simulink model "My_gfm_battery_sil_12_ConvIGBT_zDomain"  (R2025b)
settings: Solver=ode23t  StartTime=0.0  StopTime=10  MaxStep=1e-4  RelTol=1e-3
PreLoadFcn:
  | close all;
  | clear all;
  | clc;
  | 
  | 
  | modelDir = fileparts(get_param(bdroot,'FileName'));
  | 
  | load_system(fullfile(modelDir,'controls_element_lib.slx'));
  | load_system(fullfile(modelDir,'test_sequence_lib.slx'));
  | 
  | Simulink.importExternalCTypes('.\circuitControls\circuitControls_A_autogen.h')
InitFcn:
  | % frequency nominals
  | F_NOM = 60;
  | W_NOM = 2 * pi * F_NOM;
  | 
  | % base values relative to inverter
  | % --------------------------------
  | VLL_INV_NOM = 480;
  | P_INV_NOM = 1e6;
  | Q_INV_NOM = 0.5e6;
  | S_INV_NOM = sqrt(P_INV_NOM^2 + Q_INV_NOM^2);
  | 
  | I_INV_BASE = S_INV_NOM/(sqrt(3)*VLL_INV_NOM);
  | Z_INV_BASE = VLL_INV_NOM^2/S_INV_NOM;
  | L_INV_BASE = Z_INV_BASE / W_NOM;
  | C_INV_BASE = 1 / (Z_INV_BASE * W_NOM);
  | 
  | % nominal ratings for power system model
  | % --------------------------------------
  | INVERTER_COUNT = 100;
  | 
  | VLV_NOM = VLL_INV_NOM;
  | VMV_NOM = 35e3;
  | VHV_NOM = 230e3;
  | S_PLANT = INVERTER_COUNT * S_INV_NOM;
  | 
  | N_GSU = VHV_NOM/VMV_NOM;
  | N_MVT = VMV_NOM/VLV_NOM;
  | 
  | I_LV_BASE = S_PLANT/(sqrt(3)*VLV_NOM);
  | I_MV_BASE = S_PLANT/(sqrt(3)*VMV_NOM);
  | I_HV_BASE = S_PLANT/(sqrt(3)*VHV_NOM);
  | 
  | Z_LV_BASE = VLV_NOM^2/S_PLANT;
  | Z_MV_BASE = VMV_NOM^2/S_PLANT;
  | Z_HV_BASE = VHV_NOM^2/S_PLANT;
  | 
  | L_LV_BASE = Z_LV_BASE / W_NOM;
  | L_MV_BASE = Z_MV_BASE / W_NOM;
  | L_HV_BASE = Z_HV_BASE / W_NOM;
  | C_LV_BASE = 1 / (Z_LV_BASE * W_NOM);
  | C_MV_BASE = 1 / (Z_MV_BASE * W_NOM);
  | C_HV_BASE = 1 / (Z_HV_BASE * W_NOM);
undefined symbols (not defined in the file): D1, D11, Delta, gcbh, j, SampleTime, sps_rtmsupport, Ts
libraries: simulink x56, spsVoltageMeasurementLib x21, spsThreePhaseSeriesRLCBranchLib x20, spsControlledCurrentSourceLib x20, spsControlledVoltageSourceLib x15, spsThreePhaseVIMeasurementLib x12, spsSeriesRLCBranchLib x11, spsGroundLib x11, test_sequence_lib x10, controls_element_lib x8, spsCurrentMeasurementLib x8, spsThreePhaseTransformerTwoWindingsLib x6
(part 9 of 9)

== system My_gfm_battery_sil_12_ConvIGBT_zDomain/My Inverter Controller /My_machineModel_A1/governer1/LPF(DamperDecoupler) limited 1 ==
  In : Inport
  1/tau_damp : Gain  Gain=1/0.3
  Integrator : Integrator  LimitOutput=on  UpperSaturationLimit=1.2*SRated  LowerSaturationLimit=-1.2*SRated
  Sum3 : Sum  Inputs=|+-
  Out : Outport
  wires:
  Integrator/1 -> Out/1, Sum3/2
  Sum3/1 -> 1/tau_damp/1
  In/1 -> Sum3/1
  1/tau_damp/1 -> Integrator/1

== system My_gfm_battery_sil_12_ConvIGBT_zDomain/My Inverter Controller /My_machineModel_A1/governer1/synchronizer ==
  note: Why?
  note: Big Range?
  note: prevent it from acting during typical faults
  note: Prevent loss of sync at low voltage events, using asym filter to traget long extended low voltage events
  note: Keeps the machine spining in synchronize while machine is disabled, disabling the machine means
  note: Why?
  note: Should be sqrt(Vd^2 + Vq^2) ?
  Vq : Inport
  Vd : Inport  Port=2
  machine_enabled : Inport  Port=3
  Constant : Constant
  Gain : Gain  Gain=SRated
  Gain2 : Gain  Gain=1/VllRated
  HPF : Subsystem
  Product1 : Product
  Saturation : Saturate  UpperLimit=1  LowerLimit=0
  Sum : Sum  Inputs=|++
  Sum2 : Sum  Inputs=|+-
  Switch : Switch  Criteria=u2 > Threshold  SaturateOnIntegerOverflow=off  InputSameDT=off
  Transfer Fcn : TransferFcn  Commented=on  Numerator=[(2 * pi * 50) 0]  Denominator=[1, (2*pi*50)]
  assymmetric filter1 : Subsystem
  gain : Gain  Gain=2*pi*50
  kFastSync : Gain
  kSync : Gain  Gain=20
  pSyncLimit : Saturate  UpperLimit=3  LowerLimit=-3
  syncFadeGain : Gain  Gain=4
  syncFadeThreshold : Constant  Value=0.2
  to_pu : Gain  Gain=1 / VllRated
  p_sync_pu : Outport
  wires:
  to_pu/1 -> Sum2/2
  Vd/1 -> assymmetric filter1/1(in)
  assymmetric filter1/1(out) -> to_pu/1
  pSyncLimit/1 -> Gain/1
  kSync/1 -> Sum/1
  Sum/1 -> pSyncLimit/1
  Product1/1 -> p_sync_pu/1
  Constant/1 -> Switch/3
  Sum2/1 -> syncFadeGain/1
  machine_enabled/1 -> Switch/2
  syncFadeGain/1 -> Saturation/1
  Saturation/1 -> Switch/1
  syncFadeThreshold/1 -> Sum2/1
  Switch/1 -> Product1/2
  Gain2/1 -> kFastSync/1, kSync/1
  Vq/1 -> Gain2/1
  Gain/1 -> Product1/1  "p_sync"
  kFastSync/1 -> HPF/1(in)
  HPF/1(out) -> gain/1
  gain/1 -> Sum/2

== system My_gfm_battery_sil_12_ConvIGBT_zDomain/My Inverter Controller /My_machineModel_A1/rotor model/HPF (wDamperDecoupler) 1 ==
  in : Inport
  1/tau_damp : Gain  Gain=1/0.3
  Integrator : Integrator
  Sum : Sum  Inputs=|+-
  out : Outport
  wires:
  Sum/1 -> out/1, 1/tau_damp/1
  in/1 -> Sum/1
  Integrator/1 -> Sum/2
  1/tau_damp/1 -> Integrator/1

== system My_gfm_battery_sil_12_ConvIGBT_zDomain/My Inverter Controller /My_machineModel_A1/rotor model/oscillator_3ph ==
  f : Inport
  Cos : Trigonometry  Operator=cos
  Gain : Gain  Gain=2*pi
  Integrator : Integrator
  Real-Imag to Complex : RealImagToComplex
  Sin : Trigonometry
  Sum1 : Sum  Inputs=|++
  phase_shift : Constant  Value=[0 -1/3 -2/3]
  osc[3] : Outport
  wires:
  f/1 -> Integrator/1
  Real-Imag to Complex/1 -> osc[3]/1
  Cos/1 -> Real-Imag to Complex/1
  Gain/1 -> Cos/1, Sin/1
  Integrator/1 -> Sum1/1
  Sin/1 -> Real-Imag to Complex/2
  phase_shift/1 -> Sum1/2
  Sum1/1 -> Gain/1

== system My_gfm_battery_sil_12_ConvIGBT_zDomain/My Inverter Controller /My_machineModel_Other Exciter/AVR/Asym filter ==
  note: Forward integrator
  in : Inport
  Constant : Constant  Value=Ts
  Constant1 : Constant  Value=Ts
  Constant2 : Constant  Value=OmegaUp
  Constant3 : Constant  Value=OmegaUp
  Constant4 : Constant  Value=OmegaDn
  Delay : Delay  DelayLength=1  InitialCondition=0
  Product{,1..4} (5 alike) : Product
  Saturation : Saturate  UpperLimit=inf  LowerLimit=0
  Saturation1 : Saturate  UpperLimit=0  LowerLimit=-inf
  Sum : Sum  Inputs=|++
  Sum1 : Sum  Inputs=|++
  Sum4 : Sum  Inputs=|+-
  out : Outport
  wires:
  Delay/1 -> Sum4/2, Sum/2
  in/1 -> Sum4/1, Product4/2
  Sum4/1 -> Product2/1, Product1/2
  Sum/1 -> out/1, Delay/1
  Saturation/1 -> Sum1/1
  Saturation1/1 -> Sum1/2
  Sum1/1 -> Product/2
  Product/1 -> Sum/1
  Constant/1 -> Product/1
  Constant3/1 -> Product1/1
  Constant4/1 -> Product2/2
  Product1/1 -> Saturation/1
  Product2/1 -> Saturation1/1
  Product4/1 -> Product3/2
  Constant1/1 -> Product3/1
  Constant2/1 -> Product4/1

== system My_gfm_battery_sil_12_ConvIGBT_zDomain/My Inverter Controller /My_machineModel_Other Exciter/AVR/Integrator1 ==
  in : Inport
  rst : Inport  Port=2
  Constant : Constant  Value=0
  Constant1 : Constant  Value=HiLim
  Constant2 : Constant  Value=LoLim
  Constant3 : Constant  Value=Ts
  Delay : Delay  DelayLength=1  InitialCondition=0
  Logical Operator : Logic  Operator=NOT  AllPortsSameDT=off  OutDataTypeStr=boolean
  Product : Product
  Saturation Dynamic : simulink/Discontinuities/Saturation Dynamic  OutMin=[]  OutMax=[]  OutDataTypeStr=Inherit: Same as second input  OutDataType=fixdt(1, 16)  OutScaling=2^-10  DoSatur=off
  Sum : Sum  Inputs=|++
  Switch : Switch  Criteria=u2 ~= 0  SaturateOnIntegerOverflow=off  InputSameDT=off
  out : Outport
  FB : Outport  Port=2
  wires:
  Delay/1 -> Sum/2, FB/1
  Switch/1 -> Saturation Dynamic/2
  in/1 -> Product/2
  Product/1 -> Sum/1
  Constant3/1 -> Product/1
  Sum/1 -> Switch/1
  Constant/1 -> Switch/3
  rst/1 -> Logical Operator/1
  Logical Operator/1 -> Switch/2
  Saturation Dynamic/1 -> out/1, Delay/1
  Constant1/1 -> Saturation Dynamic/1
  Constant2/1 -> Saturation Dynamic/3

== system My_gfm_battery_sil_12_ConvIGBT_zDomain/My Inverter Controller /My_machineModel_Other Exciter/AVR/Q LPF ==
  note: Forward integrator
  in : Inport
  Constant : Constant  Value=Ts
  Constant1 : Constant  Value=Ts
  Constant2 : Constant  Value=OmegaUp
  Constant3 : Constant  Value=OmegaUp
  Constant4 : Constant  Value=OmegaDn
  Delay : Delay  DelayLength=1  InitialCondition=0
  Product{,1..4} (5 alike) : Product
  Saturation : Saturate  UpperLimit=inf  LowerLimit=0
  Saturation1 : Saturate  UpperLimit=0  LowerLimit=-inf
  Sum : Sum  Inputs=|++
  Sum1 : Sum  Inputs=|++
  Sum4 : Sum  Inputs=|+-
  out : Outport
  wires:
  Delay/1 -> Sum4/2, Sum/2
  in/1 -> Sum4/1, Product4/2
  Sum4/1 -> Product2/1, Product1/2
  Sum/1 -> out/1, Delay/1
  Saturation/1 -> Sum1/1
  Saturation1/1 -> Sum1/2
  Sum1/1 -> Product/2
  Product/1 -> Sum/1
  Constant/1 -> Product/1
  Constant3/1 -> Product1/1
  Constant4/1 -> Product2/2
  Product1/1 -> Saturation/1
  Product2/1 -> Saturation1/1
  Product4/1 -> Product3/2
  Constant1/1 -> Product3/1
  Constant2/1 -> Product4/1

== system My_gfm_battery_sil_12_ConvIGBT_zDomain/My Inverter Controller /My_machineModel_Other Exciter/AVR/V LPF ==
  note: Forward integrator
  in : Inport
  Constant : Constant  Value=Ts
  Constant1 : Constant  Value=Ts
  Constant2 : Constant  Value=OmegaUp
  Constant3 : Constant  Value=OmegaUp
  Constant4 : Constant  Value=OmegaDn
  Delay : Delay  DelayLength=1  InitialCondition=0
  Product{,1..4} (5 alike) : Product
  Saturation : Saturate  UpperLimit=inf  LowerLimit=0
  Saturation1 : Saturate  UpperLimit=0  LowerLimit=-inf
  Sum : Sum  Inputs=|++
  Sum1 : Sum  Inputs=|++
  Sum4 : Sum  Inputs=|+-
  out : Outport
  wires:
  Delay/1 -> Sum4/2, Sum/2
  in/1 -> Sum4/1, Product4/2
  Sum4/1 -> Product2/1, Product1/2
  Sum/1 -> out/1, Delay/1
  Saturation/1 -> Sum1/1
  Saturation1/1 -> Sum1/2
  Sum1/1 -> Product/2
  Product/1 -> Sum/1
  Constant/1 -> Product/1
  Constant3/1 -> Product1/1
  Constant4/1 -> Product2/2
  Product1/1 -> Saturation/1
  Product2/1 -> Saturation1/1
  Product4/1 -> Product3/2
  Constant1/1 -> Product3/1
  Constant2/1 -> Product4/1

== system My_gfm_battery_sil_12_ConvIGBT_zDomain/My Inverter Controller /My_machineModel_Other Exciter/Exciter/LPF4 ==
  note: Forward integrator
  in : Inport
  Constant : Constant  Value=Ts
  Constant1 : Constant  Value=Ts
  Constant2 : Constant  Value=OmegaUp
  Constant3 : Constant  Value=OmegaUp
  Constant4 : Constant  Value=OmegaDn
  Delay : Delay  DelayLength=1  InitialCondition=0
  Product{,1..4} (5 alike) : Product
  Saturation : Saturate  UpperLimit=inf  LowerLimit=0
  Saturation1 : Saturate  UpperLimit=0  LowerLimit=-inf
  Sum : Sum  Inputs=|++
  Sum1 : Sum  Inputs=|++
  Sum4 : Sum  Inputs=|+-
  out : Outport
  wires:
  Delay/1 -> Sum4/2, Sum/2
  in/1 -> Sum4/1, Product4/2
  Sum4/1 -> Product2/1, Product1/2
  Sum/1 -> out/1, Delay/1
  Saturation/1 -> Sum1/1
  Saturation1/1 -> Sum1/2
  Sum1/1 -> Product/2
  Product/1 -> Sum/1
  Constant/1 -> Product/1
  Constant3/1 -> Product1/1
  Constant4/1 -> Product2/2
  Product1/1 -> Saturation/1
  Product2/1 -> Saturation1/1
  Product4/1 -> Product3/2
  Constant1/1 -> Product3/1
  Constant2/1 -> Product4/1

== system My_gfm_battery_sil_12_ConvIGBT_zDomain/My Inverter Controller /My_machineModel_Other Exciter/Exciter/modulator ==
  cmd : Inport
  osc : Inport  Port=2
  Complex to Real-Imag : ComplexToRealImag
  Complex to Real-Imag1 : ComplexToRealImag
  Gain : Gain  Gain=sqrt(2)
  Product1 : Product
  Product2 : Product
  Sum1 : Sum  Inputs=|+-
  ref : Outport
  wires:
  osc/1 -> Gain/1
  Complex to Real-Imag/1 -> Product2/2
  Product2/1 -> Sum1/1
  Sum1/1 -> ref/1  "i"
  Gain/1 -> Complex to Real-Imag/1
  Complex to Real-Imag/2 -> Product1/2
  Product1/1 -> Sum1/2
  cmd/1 -> Complex to Real-Imag1/1
  Complex to Real-Imag1/1 -> Product2/1
  Complex to Real-Imag1/2 -> Product1/1

== system My_gfm_battery_sil_12_ConvIGBT_zDomain/My Inverter Controller /My_machineModel_Other Exciter/governer/LPF(DamperDecoupler) limited  ==
  note: Forward integrator
  in : Inport
  Constant : Constant  Value=Ts
  Constant1 : Constant  Value=0
  Constant2 : Constant  Value=DnLim
  Constant3 : Constant  Value=OmegaUp
  Constant4 : Constant  Value=OmegaDn
  Constant5 : Constant  Value=UpLim
  Constant6 : Constant  Value=0
  Delay : Delay  DelayLength=1  InitialCondition=0
  Product : Product
  Product1 : Product
  Product2 : Product
  Saturation Dynamic1 : simulink/Discontinuities/Saturation Dynamic  OutMin=[]  OutMax=[]  OutDataTypeStr=Inherit: Same as second input  OutDataType=fixdt(1, 16)  OutScaling=2^-10  DoSatur=off
  Saturation Dynamic2 : simulink/Discontinuities/Saturation Dynamic  OutMin=[]  OutMax=[]  OutDataTypeStr=Inherit: Same as second input  OutDataType=fixdt(1, 16)  OutScaling=2^-10  DoSatur=off
  Sum : Sum  Inputs=|++
  Sum1 : Sum  Inputs=|++
  Sum4 : Sum  Inputs=|+-
  out : Outport
  wires:
  Delay/1 -> Sum/2, Sum4/2
  in/1 -> Sum4/1
  Sum4/1 -> Product2/1, Product1/2
  Sum/1 -> out/1, Delay/1
  Product/1 -> Sum/1
  Constant/1 -> Product/1
  Constant3/1 -> Product1/1
  Constant4/1 -> Product2/2
  Sum1/1 -> Product/2
  Constant6/1 -> Saturation Dynamic1/3
  Product1/1 -> Saturation Dynamic1/2
  Constant5/1 -> Saturation Dynamic1/1
  Saturation Dynamic1/1 -> Sum1/1
  Constant1/1 -> Saturation Dynamic2/1
  Product2/1 -> Saturation Dynamic2/2
  Constant2/1 -> Saturation Dynamic2/3
  Saturation Dynamic2/1 -> Sum1/2

== system My_gfm_battery_sil_12_ConvIGBT_zDomain/My Inverter Controller /My_machineModel_Other Exciter/governer/synchronizer ==
  note: Big Range?
  note: prevent it from acting during typical faults
  note: Prevent loss of sync at low voltage events, using asym filter to traget long extended low voltage events
  note: Keeps the machine spining in synchronize while machine is disabled, disabling the machine means
  note: Why?
  Vq : Inport
  Vt : Inport  Port=2
  machine_enabled : Inport  Port=3
  Asym filter : Subsystem  SystemSampleTime=0.001  mask(Low Pass Filter){Ts=Ts, OmegaUp=1/tauBkSt, OmegaDn=0.01/tauBkSt, UpLim=inf, DnLim=-inf}
      mask prompts: Ts "Tsample"; OmegaUp "Up Path Bandwidth"; OmegaDn "Down Path Bandwidth"; UpLim "Up Limiter"; DnLim "Down Limiter"
  Constant : Constant
  Damping HPF : Subsystem  mask(High Pass Filter){Ts=Ts, OmegaUp=wSync, OmegaDn=wSync}
      mask prompts: Ts "Tsample"; OmegaUp "Up Path Bandwidth"; OmegaDn "Down Path Bandwidth"
      mask help: Min. Tsample is 1/20000; Max. Omega is 0.2/Ts
      mask DialogControl Container2 Prompt: Parameters
  Gain : Gain  Gain=SRated
  Gain2 : Gain  Gain=1/VllRated
  Product1 : Product
  Saturation : Saturate  UpperLimit=1  LowerLimit=0
  Sum : Sum  Inputs=|++
  Sum2 : Sum  Inputs=|+-
  Switch : Switch  Criteria=u2 > Threshold  SaturateOnIntegerOverflow=off  InputSameDT=off
  gain : Gain  Gain=wSync
  kFastSync : Gain  Gain=kpFastSync
  kSync : Gain  Gain=kpSync
  pSyncLimit : Saturate  UpperLimit=3  LowerLimit=-3
  syncFadeGain : Gain  Gain=kpSyncFade
  syncFadeThreshold : Constant  Value=SyncFadeThres
  to_pu : Gain  Gain=1 / VllRated
  p_sync_pu : Outport
  wires:
  to_pu/1 -> Sum2/2
  Vt/1 -> Asym filter/1(in)
  Asym filter/1(out) -> to_pu/1
  pSyncLimit/1 -> Gain/1
  kSync/1 -> Sum/1
  Sum/1 -> pSyncLimit/1
  Product1/1 -> p_sync_pu/1
  Constant/1 -> Switch/3
  Sum2/1 -> syncFadeGain/1
  machine_enabled/1 -> Switch/2
  syncFadeGain/1 -> Saturation/1
  Saturation/1 -> Switch/1
  syncFadeThreshold/1 -> Sum2/1
  Switch/1 -> Product1/2
  Gain2/1 -> kFastSync/1, kSync/1
  Vq/1 -> Gain2/1
  Gain/1 -> Product1/1  "p_sync"
  kFastSync/1 -> Damping HPF/1(in)
  gain/1 -> Sum/2
  Damping HPF/1(out) -> gain/1

== system My_gfm_battery_sil_12_ConvIGBT_zDomain/My Inverter Controller /My_machineModel_Other Exciter/impedance emulation/Integrator1 ==
  in : Inport
  rst : Inport  Port=2
  Constant : Constant  Value=0
  Constant1 : Constant  Value=HiLim
  Constant2 : Constant  Value=LoLim
  Constant3 : Constant  Value=Ts
  Delay : Delay  DelayLength=1  InitialCondition=0
  Logical Operator : Logic  Operator=NOT  AllPortsSameDT=off  OutDataTypeStr=boolean
  Product : Product
  Saturation Dynamic : simulink/Discontinuities/Saturation Dynamic  OutMin=[]  OutMax=[]  OutDataTypeStr=Inherit: Same as second input  OutDataType=fixdt(1, 16)  OutScaling=2^-10  DoSatur=off
  Sum : Sum  Inputs=|++
  Switch : Switch  Criteria=u2 ~= 0  SaturateOnIntegerOverflow=off  InputSameDT=off
  out : Outport
  FB : Outport  Port=2
  wires:
  Delay/1 -> Sum/2, FB/1
  Switch/1 -> Saturation Dynamic/2
  in/1 -> Product/2
  Product/1 -> Sum/1
  Constant3/1 -> Product/1
  Sum/1 -> Switch/1
  Constant/1 -> Switch/3
  rst/1 -> Logical Operator/1
  Logical Operator/1 -> Switch/2
  Saturation Dynamic/1 -> out/1, Delay/1
  Constant1/1 -> Saturation Dynamic/1
  Constant2/1 -> Saturation Dynamic/3

== system My_gfm_battery_sil_12_ConvIGBT_zDomain/My Inverter Controller /My_machineModel_Other Exciter/rotor model/Damping HPF ==
  note: Forward integrator
  in : Inport
  Constant2 : Constant  Value=Ts
  Constant3 : Constant  Value=OmegaUp
  Constant4 : Constant  Value=OmegaDn
  Delay : Delay  DelayLength=1  InitialCondition=0
  Product : Product
  Product1 : Product
  Product2 : Product
  Saturation : Saturate  UpperLimit=inf  LowerLimit=0
  Saturation1 : Saturate  UpperLimit=0  LowerLimit=-inf
  Sum : Sum  Inputs=|+-
  Sum1 : Sum  Inputs=|++
  Sum2 : Sum  Inputs=|++
  Sum3 : Sum  Inputs=|+-
  out : Outport  VectorParamsAs1DForOutWhenUnconnected=off
  wires:
  Delay/1 -> Sum1/2, Sum/2
  Sum/1 -> Product2/1, Product1/2
  Saturation/1 -> Sum2/1
  Sum1/1 -> Sum3/2, Delay/1
  Sum2/1 -> Product/2
  Product/1 -> Sum1/1
  Product2/1 -> Saturation1/1
  in/1 -> Sum3/1, Sum/1
  Product1/1 -> Saturation/1
  Saturation1/1 -> Sum2/2
  Sum3/1 -> out/1
  Constant2/1 -> Product/1
  Constant3/1 -> Product1/1
  Constant4/1 -> Product2/2

== system My_gfm_battery_sil_12_ConvIGBT_zDomain/My Inverter Controller /My_machineModel_Other Exciter/rotor model/Integrator ==
  in : Inport
  rst : Inport  Port=2
  Constant : Constant  Value=0
  Constant1 : Constant  Value=HiLim
  Constant2 : Constant  Value=LoLim
  Constant3 : Constant  Value=Ts
  Delay : Delay  DelayLength=1  InitialCondition=0
  Logical Operator : Logic  Operator=NOT  AllPortsSameDT=off  OutDataTypeStr=boolean
  Product : Product
  Saturation Dynamic : simulink/Discontinuities/Saturation Dynamic  OutMin=[]  OutMax=[]  OutDataTypeStr=Inherit: Same as second input  OutDataType=fixdt(1, 16)  OutScaling=2^-10  DoSatur=off
  Sum : Sum  Inputs=|++
  Switch : Switch  Criteria=u2 ~= 0  SaturateOnIntegerOverflow=off  InputSameDT=off
  out : Outport
  FB : Outport  Port=2
  wires:
  Delay/1 -> Sum/2, FB/1
  Switch/1 -> Saturation Dynamic/2
  in/1 -> Product/2
  Product/1 -> Sum/1
  Constant3/1 -> Product/1
  Sum/1 -> Switch/1
  Constant/1 -> Switch/3
  rst/1 -> Logical Operator/1
  Logical Operator/1 -> Switch/2
  Saturation Dynamic/1 -> out/1, Delay/1
  Constant1/1 -> Saturation Dynamic/1
  Constant2/1 -> Saturation Dynamic/3

== system My_gfm_battery_sil_12_ConvIGBT_zDomain/My Inverter Controller /My_machineModel_Other Exciter/rotor model/oscillator_3ph ==
  f : Inport
  Cos : Trigonometry  Operator=cos
  Delay : Delay  DelayLength=1  InitialCondition=0
  Gain : Gain  Gain=2*pi
  Ground1 : Ground
  Integrator : Subsystem  SystemSampleTime=1/20000  mask(Wrapped Integrator){Ts=Ts}
      mask prompts: Ts "Tsample"
      mask help: output range : [0 to 1]
  Real-Imag to Complex : RealImagToComplex
  Scope : Scope
      settings: ActiveDisplayYMinimum=-0.026446027315415011  ActiveDisplayYMaximum=1.0606778639513765  DataLoggingVariableName=ScopeData13
  Sin : Trigonometry
  Sum1 : Sum  Inputs=|++
  Terminator : Terminator
  phase_shift : Constant  Value=[0 -1/3 -2/3]
  osc[3] : Outport
  osc[3]_FB : Outport  Port=2
  wires:
  Sum1/1 -> Gain/1
  phase_shift/1 -> Sum1/2
  Sin/1 -> Real-Imag to Complex/2
  Gain/1 -> Sin/1, Cos/1
  Cos/1 -> Real-Imag to Complex/1
  Real-Imag to Complex/1 -> Delay/1, osc[3]/1
  f/1 -> Integrator/1(in)
  Delay/1 -> osc[3]_FB/1
  Integrator/2(FB) -> Terminator/1
  Ground1/1 -> Integrator/2(rst)
  Integrator/1(out) -> Scope/1, Sum1/1

== system My_gfm_battery_sil_12_ConvIGBT_zDomain/My Inverter Controller /My_machineModel_Other Exciter/voltage analyzer/LPF ==
  note: Forward integrator
  in : Inport
  Constant : Constant  Value=Ts
  Constant1 : Constant  Value=Ts
  Constant2 : Constant  Value=OmegaUp
  Constant3 : Constant  Value=OmegaUp
  Constant4 : Constant  Value=OmegaDn
  Delay : Delay  DelayLength=1  InitialCondition=0
  Product{,1..4} (5 alike) : Product
  Saturation : Saturate  UpperLimit=inf  LowerLimit=0
  Saturation1 : Saturate  UpperLimit=0  LowerLimit=-inf
  Sum : Sum  Inputs=|++
  Sum1 : Sum  Inputs=|++
  Sum4 : Sum  Inputs=|+-
  out : Outport
  wires:
  Delay/1 -> Sum4/2, Sum/2
  in/1 -> Sum4/1, Product4/2
  Sum4/1 -> Product2/1, Product1/2
  Sum/1 -> out/1, Delay/1
  Saturation/1 -> Sum1/1
  Saturation1/1 -> Sum1/2
  Sum1/1 -> Product/2
  Product/1 -> Sum/1
  Constant/1 -> Product/1
  Constant3/1 -> Product1/1
  Constant4/1 -> Product2/2
  Product1/1 -> Saturation/1
  Product2/1 -> Saturation1/1
  Product4/1 -> Product3/2
  Constant1/1 -> Product3/1
  Constant2/1 -> Product4/1

== system My_gfm_battery_sil_12_ConvIGBT_zDomain/My Inverter Controller /My_machineModel_Other Exciter/voltage analyzer/LPF1 ==
  note: Forward integrator
  in : Inport
  Constant : Constant  Value=Ts
  Constant1 : Constant  Value=Ts
  Constant2 : Constant  Value=OmegaUp
  Constant3 : Constant  Value=OmegaUp
  Constant4 : Constant  Value=OmegaDn
  Delay : Delay  DelayLength=1  InitialCondition=0
  Product{,1..4} (5 alike) : Product
  Saturation : Saturate  UpperLimit=inf  LowerLimit=0
  Saturation1 : Saturate  UpperLimit=0  LowerLimit=-inf
  Sum : Sum  Inputs=|++
  Sum1 : Sum  Inputs=|++
  Sum4 : Sum  Inputs=|+-
  out : Outport
  wires:
  Delay/1 -> Sum4/2, Sum/2
  in/1 -> Sum4/1, Product4/2
  Sum4/1 -> Product2/1, Product1/2
  Sum/1 -> out/1, Delay/1
  Saturation/1 -> Sum1/1
  Saturation1/1 -> Sum1/2
  Sum1/1 -> Product/2
  Product/1 -> Sum/1
  Constant/1 -> Product/1
  Constant3/1 -> Product1/1
  Constant4/1 -> Product2/2
  Product1/1 -> Saturation/1
  Product2/1 -> Saturation1/1
  Product4/1 -> Product3/2
  Constant1/1 -> Product3/1
  Constant2/1 -> Product4/1

== system My_gfm_battery_sil_12_ConvIGBT_zDomain/Plant controller (simplified example)/Meter/PLL-analog/oscillator_3ph ==
  f : Inport
  Cos : Trigonometry  Operator=cos
  Gain : Gain  Gain=2*pi
  Integrator : Integrator
  Real-Imag to Complex : RealImagToComplex
  Sin : Trigonometry
  Sum1 : Sum  Inputs=|++
  phase_shift : Constant  Value=[0 -1/3 -2/3]
  osc[3] : Outport
  wires:
  Sum1/1 -> Gain/1
  phase_shift/1 -> Sum1/2
  Sin/1 -> Real-Imag to Complex/2
  Integrator/1 -> Sum1/1
  Gain/1 -> Sin/1, Cos/1
  Cos/1 -> Real-Imag to Complex/1
  Real-Imag to Complex/1 -> osc[3]/1
  f/1 -> Integrator/1

== system My_gfm_battery_sil_12_ConvIGBT_zDomain/My Inverter Controller /My_acMonitor_A/Analyzer_V/complex_LPF/LPF1 ==
  note: Forward integrator
  in : Inport
  Constant : Constant  Value=Ts
  Constant1 : Constant  Value=Ts
  Constant2 : Constant  Value=OmegaUp
  Constant3 : Constant  Value=OmegaUp
  Constant4 : Constant  Value=OmegaDn
  Delay : Delay  DelayLength=1  InitialCondition=0
  Product{,1..4} (5 alike) : Product
  Saturation : Saturate  UpperLimit=inf  LowerLimit=0
  Saturation1 : Saturate  UpperLimit=0  LowerLimit=-inf
  Sum : Sum  Inputs=|++
  Sum1 : Sum  Inputs=|++
  Sum4 : Sum  Inputs=|+-
  out : Outport
  wires:
  Delay/1 -> Sum4/2, Sum/2
  in/1 -> Sum4/1, Product4/2
  Sum4/1 -> Product2/1, Product1/2
  Sum/1 -> out/1, Delay/1
  Saturation/1 -> Sum1/1
  Saturation1/1 -> Sum1/2
  Sum1/1 -> Product/2
  Product/1 -> Sum/1
  Constant/1 -> Product/1
  Constant3/1 -> Product1/1
  Constant4/1 -> Product2/2
  Product1/1 -> Saturation/1
  Product2/1 -> Saturation1/1
  Product4/1 -> Product3/2
  Constant1/1 -> Product3/1
  Constant2/1 -> Product4/1

== system My_gfm_battery_sil_12_ConvIGBT_zDomain/My Inverter Controller /My_acMonitor_A/Analyzer_V/complex_LPF/LPF4 ==
  note: Forward integrator
  in : Inport
  Constant : Constant  Value=Ts
  Constant1 : Constant  Value=Ts
  Constant2 : Constant  Value=OmegaUp
  Constant3 : Constant  Value=OmegaUp
  Constant4 : Constant  Value=OmegaDn
  Delay : Delay  DelayLength=1  InitialCondition=0
  Product{,1..4} (5 alike) : Product
  Saturation : Saturate  UpperLimit=inf  LowerLimit=0
  Saturation1 : Saturate  UpperLimit=0  LowerLimit=-inf
  Sum : Sum  Inputs=|++
  Sum1 : Sum  Inputs=|++
  Sum4 : Sum  Inputs=|+-
  Terminator : Terminator
  out : Outport
  wires:
  Delay/1 -> Sum4/2, Sum/2
  in/1 -> Sum4/1, Product4/2
  Sum4/1 -> Product2/1, Product1/2
  Sum/1 -> out/1, Delay/1
  Saturation/1 -> Sum1/1
  Saturation1/1 -> Sum1/2
  Sum1/1 -> Product/2
  Product/1 -> Sum/1
  Constant/1 -> Product/1
  Constant3/1 -> Product1/1
  Constant4/1 -> Product2/2
  Product1/1 -> Saturation/1
  Product2/1 -> Saturation1/1
  Product4/1 -> Product3/2
  Constant1/1 -> Product3/1
  Constant2/1 -> Product4/1
  Product3/1 -> Terminator/1

== system My_gfm_battery_sil_12_ConvIGBT_zDomain/My Inverter Controller /My_acMonitor_A/PLL_3ph1/SOGI1/Integrator ==
  in : Inport
  rst : Inport  Port=2
  Constant : Constant  Value=0
  Constant1 : Constant  Value=HiLim
  Constant2 : Constant  Value=LoLim
  Constant3 : Constant  Value=Ts
  Delay : Delay  DelayLength=1  InitialCondition=0
  Logical Operator : Logic  Operator=NOT  AllPortsSameDT=off  OutDataTypeStr=boolean
  Product : Product
  Saturation Dynamic : simulink/Discontinuities/Saturation Dynamic  OutMin=[]  OutMax=[]  OutDataTypeStr=Inherit: Same as second input  OutDataType=fixdt(1, 16)  OutScaling=2^-10  DoSatur=off
  Sum : Sum  Inputs=|++
  Switch : Switch  Criteria=u2 ~= 0  SaturateOnIntegerOverflow=off  InputSameDT=off
  out : Outport
  FB : Outport  Port=2
  wires:
  Delay/1 -> Sum/2, FB/1
  Switch/1 -> Saturation Dynamic/2
  in/1 -> Product/2
  Product/1 -> Sum/1
  Constant3/1 -> Product/1
  Sum/1 -> Switch/1
  Constant/1 -> Switch/3
  rst/1 -> Logical Operator/1
  Logical Operator/1 -> Switch/2
  Saturation Dynamic/1 -> out/1, Delay/1
  Constant1/1 -> Saturation Dynamic/1
  Constant2/1 -> Saturation Dynamic/3

== system My_gfm_battery_sil_12_ConvIGBT_zDomain/My Inverter Controller /My_acMonitor_A/PLL_3ph1/SOGI1/Integrator1 ==
  in : Inport
  rst : Inport  Port=2
  Constant : Constant  Value=0
  Constant1 : Constant  Value=HiLim
  Constant2 : Constant  Value=LoLim
  Constant3 : Constant  Value=Ts
  Delay : Delay  DelayLength=1  InitialCondition=0
  Logical Operator : Logic  Operator=NOT  AllPortsSameDT=off  OutDataTypeStr=boolean
  Product : Product
  Saturation Dynamic : simulink/Discontinuities/Saturation Dynamic  OutMin=[]  OutMax=[]  OutDataTypeStr=Inherit: Same as second input  OutDataType=fixdt(1, 16)  OutScaling=2^-10  DoSatur=off
  Sum : Sum  Inputs=|++
  Switch : Switch  Criteria=u2 ~= 0  SaturateOnIntegerOverflow=off  InputSameDT=off
  out : Outport
  FB : Outport  Port=2
  wires:
  Delay/1 -> Sum/2, FB/1
  Switch/1 -> Saturation Dynamic/2
  in/1 -> Product/2
  Product/1 -> Sum/1
  Constant3/1 -> Product/1
  Sum/1 -> Switch/1
  Constant/1 -> Switch/3
  rst/1 -> Logical Operator/1
  Logical Operator/1 -> Switch/2
  Saturation Dynamic/1 -> out/1, Delay/1
  Constant1/1 -> Saturation Dynamic/1
  Constant2/1 -> Saturation Dynamic/3

== system My_gfm_battery_sil_12_ConvIGBT_zDomain/My Inverter Controller /My_acMonitor_A/PLL_3ph1/oscillator_3ph/Integrator ==
  in : Inport
  rst : Inport  Port=2
  Constant : Constant  Value=0
  Constant1 : Constant  Value=Ts
  Delay : Delay  DelayLength=1  InitialCondition=0
  Logical Operator : Logic  Operator=NOT  AllPortsSameDT=off  OutDataTypeStr=boolean
  Product : Product
  Rounding Function : Rounding
  Sum : Sum  Inputs=|++
  Sum1 : Sum  Inputs=|+-
  Switch : Switch  Criteria=u2 ~= 0  SaturateOnIntegerOverflow=off  InputSameDT=off
  out : Outport
  FB : Outport  Port=2
  wires:
  Delay/1 -> Sum/2, FB/1
  in/1 -> Product/2
  Product/1 -> Sum/1
  Constant1/1 -> Product/1
  Sum/1 -> Switch/1
  Constant/1 -> Switch/3
  rst/1 -> Logical Operator/1
  Logical Operator/1 -> Switch/2
  Switch/1 -> Sum1/1, Rounding Function/1
  Rounding Function/1 -> Sum1/2
  Sum1/1 -> Delay/1, out/1

== system My_gfm_battery_sil_12_ConvIGBT_zDomain/My Inverter Controller /My_machineModel_A1/governer/synchronizer/HPF ==
  in : Inport
  1/tau : Gain  Gain=2*pi*50
  Integrator : Integrator
  Sum : Sum  Inputs=|+-
  out : Outport
  wires:
  Sum/1 -> out/1, 1/tau/1
  in/1 -> Sum/1
  Integrator/1 -> Sum/2
  1/tau/1 -> Integrator/1

== system My_gfm_battery_sil_12_ConvIGBT_zDomain/My Inverter Controller /My_machineModel_A1/governer/synchronizer/assymmetric filter1 ==
  note: The saturation block is configured to cause a rapid rise, but much slow drop in output.
  in : Inport
  Gain1 : Gain  Gain=2
  Integrator : Integrator
  Saturation1 : Saturate  UpperLimit=VllRated  LowerLimit=-0.02 * VllRated
  Sum3 : Sum  Inputs=|+-
  out : Outport
  wires:
  Integrator/1 -> out/1, Sum3/2
  Sum3/1 -> Gain1/1
  in/1 -> Sum3/1
  Gain1/1 -> Saturation1/1
  Saturation1/1 -> Integrator/1

== system My_gfm_battery_sil_12_ConvIGBT_zDomain/My Inverter Controller /My_machineModel_A1/governer1/synchronizer/HPF ==
  in : Inport
  1/tau : Gain  Gain=2*pi*50
  Integrator : Integrator
  Sum : Sum  Inputs=|+-
  out : Outport
  wires:
  Sum/1 -> out/1, 1/tau/1
  in/1 -> Sum/1
  Integrator/1 -> Sum/2
  1/tau/1 -> Integrator/1

== system My_gfm_battery_sil_12_ConvIGBT_zDomain/My Inverter Controller /My_machineModel_A1/governer1/synchronizer/assymmetric filter1 ==
  note: The saturation block is configured to cause a rapid rise, but much slow drop in output.
  in : Inport
  Gain1 : Gain  Gain=2
  Integrator : Integrator
  Saturation1 : Saturate  UpperLimit=VllRated  LowerLimit=-0.02 * VllRated
  Sum3 : Sum  Inputs=|+-
  out : Outport
  wires:
  Integrator/1 -> out/1, Sum3/2
  Sum3/1 -> Gain1/1
  in/1 -> Sum3/1
  Gain1/1 -> Saturation1/1
  Saturation1/1 -> Integrator/1

== system My_gfm_battery_sil_12_ConvIGBT_zDomain/My Inverter Controller /My_machineModel_Other Exciter/governer/synchronizer/Asym filter ==
  note: Forward integrator
  in : Inport
  Constant : Constant  Value=Ts
  Constant1 : Constant  Value=0
  Constant2 : Constant  Value=DnLim
  Constant3 : Constant  Value=OmegaUp
  Constant4 : Constant  Value=OmegaDn
  Constant5 : Constant  Value=UpLim
  Constant6 : Constant  Value=0
  Delay : Delay  DelayLength=1  InitialCondition=0
  Product : Product
  Product1 : Product
  Product2 : Product
  Saturation Dynamic1 : simulink/Discontinuities/Saturation Dynamic  OutMin=[]  OutMax=[]  OutDataTypeStr=Inherit: Same as second input  OutDataType=fixdt(1, 16)  OutScaling=2^-10  DoSatur=off
  Saturation Dynamic2 : simulink/Discontinuities/Saturation Dynamic  OutMin=[]  OutMax=[]  OutDataTypeStr=Inherit: Same as second input  OutDataType=fixdt(1, 16)  OutScaling=2^-10  DoSatur=off
  Sum : Sum  Inputs=|++
  Sum1 : Sum  Inputs=|++
  Sum4 : Sum  Inputs=|+-
  out : Outport
  wires:
  Delay/1 -> Sum/2, Sum4/2
  in/1 -> Sum4/1
  Sum4/1 -> Product2/1, Product1/2
  Sum/1 -> out/1, Delay/1
  Product/1 -> Sum/1
  Constant/1 -> Product/1
  Constant3/1 -> Product1/1
  Constant4/1 -> Product2/2
  Sum1/1 -> Product/2
  Constant6/1 -> Saturation Dynamic1/3
  Product1/1 -> Saturation Dynamic1/2
  Constant5/1 -> Saturation Dynamic1/1
  Saturation Dynamic1/1 -> Sum1/1
  Constant1/1 -> Saturation Dynamic2/1
  Product2/1 -> Saturation Dynamic2/2
  Constant2/1 -> Saturation Dynamic2/3
  Saturation Dynamic2/1 -> Sum1/2

== system My_gfm_battery_sil_12_ConvIGBT_zDomain/My Inverter Controller /My_machineModel_Other Exciter/governer/synchronizer/Damping HPF ==
  note: Forward integrator
  in : Inport
  Constant2 : Constant  Value=Ts
  Constant3 : Constant  Value=OmegaUp
  Constant4 : Constant  Value=OmegaDn
  Delay : Delay  DelayLength=1  InitialCondition=0
  Product : Product
  Product1 : Product
  Product2 : Product
  Saturation : Saturate  UpperLimit=inf  LowerLimit=0
  Saturation1 : Saturate  UpperLimit=0  LowerLimit=-inf
  Sum : Sum  Inputs=|+-
  Sum1 : Sum  Inputs=|++
  Sum2 : Sum  Inputs=|++
  Sum3 : Sum  Inputs=|+-
  out : Outport  VectorParamsAs1DForOutWhenUnconnected=off
  wires:
  Delay/1 -> Sum1/2, Sum/2
  Sum/1 -> Product2/1, Product1/2
  Saturation/1 -> Sum2/1
  Sum1/1 -> Sum3/2, Delay/1
  Sum2/1 -> Product/2
  Product/1 -> Sum1/1
  Product2/1 -> Saturation1/1
  in/1 -> Sum3/1, Sum/1
  Product1/1 -> Saturation/1
  Saturation1/1 -> Sum2/2
  Sum3/1 -> out/1
  Constant2/1 -> Product/1
  Constant3/1 -> Product1/1
  Constant4/1 -> Product2/2

== system My_gfm_battery_sil_12_ConvIGBT_zDomain/My Inverter Controller /My_machineModel_Other Exciter/rotor model/oscillator_3ph/Integrator ==
  in : Inport
  rst : Inport  Port=2
  Constant : Constant  Value=0
  Constant1 : Constant  Value=Ts
  Delay : Delay  DelayLength=1  InitialCondition=0
  Logical Operator : Logic  Operator=NOT  AllPortsSameDT=off  OutDataTypeStr=boolean
  Product : Product
  Rounding Function : Rounding
  Sum : Sum  Inputs=|++
  Sum1 : Sum  Inputs=|+-
  Switch : Switch  Criteria=u2 ~= 0  SaturateOnIntegerOverflow=off  InputSameDT=off
  out : Outport
  FB : Outport  Port=2
  wires:
  Delay/1 -> Sum/2, FB/1
  in/1 -> Product/2
  Product/1 -> Sum/1
  Constant1/1 -> Product/1
  Sum/1 -> Switch/1
  Constant/1 -> Switch/3
  rst/1 -> Logical Operator/1
  Logical Operator/1 -> Switch/2
  Switch/1 -> Sum1/1, Rounding Function/1
  Rounding Function/1 -> Sum1/2
  Sum1/1 -> Delay/1, out/1

== matlab function My_gfm_battery_sil_12_ConvIGBT_zDomain/ac Network with MVT (native math)5/Two-Level Converter/Model1/MATLAB Function ==
  data: g input; V output; Vdc input; I input; Idc output
function [V,Idc] = FunctionHalfBridge1(g,Vdc,I)
[V,Idc]=FunctionHalfBridge(g,Vdc,I);

== matlab function My_gfm_battery_sil_12_ConvIGBT_zDomain/ac Network with MVT (native math)5/Two-Level Converter/Model2/MATLAB Function ==
  data: g input; V output; Vdc input; I input; Idc output
function [V,Idc] = FunctionHalfBridge1(g,Vdc,I)
[V,Idc]=FunctionHalfBridge(g,Vdc,I);

== matlab function My_gfm_battery_sil_12_ConvIGBT_zDomain/ac Network with MVT (native math)5/Two-Level Converter/Model3/MATLAB Function ==
  data: g input; V output; Vdc input; I input; Idc output
function [V,Idc] = FunctionHalfBridge1(g,Vdc,I)
[V,Idc]=FunctionHalfBridge(g,Vdc,I);

== matlab function My_gfm_battery_sil_12_ConvIGBT_zDomain/ac Network with MVT (native math)4/Two-Level Converter/Model1/MATLAB Function ==
  data: g input; V output; Vdc input; I input; Idc output
function [V,Idc] = FunctionHalfBridge1(g,Vdc,I)
[V,Idc]=FunctionHalfBridge(g,Vdc,I);

== matlab function My_gfm_battery_sil_12_ConvIGBT_zDomain/ac Network with MVT (native math)4/Two-Level Converter/Model2/MATLAB Function ==
  data: g input; V output; Vdc input; I input; Idc output
function [V,Idc] = FunctionHalfBridge1(g,Vdc,I)
[V,Idc]=FunctionHalfBridge(g,Vdc,I);

== matlab function My_gfm_battery_sil_12_ConvIGBT_zDomain/ac Network with MVT (native math)4/Two-Level Converter/Model3/MATLAB Function ==
  data: g input; V output; Vdc input; I input; Idc output
function [V,Idc] = FunctionHalfBridge1(g,Vdc,I)
[V,Idc]=FunctionHalfBridge(g,Vdc,I);
